simulink model "Copy_of_sistema_angulo"  (R2024b)
settings: Solver=ode4  StartTime=0.0  StopTime=tfin+ts  FixedStep=ts  MaxStep=ts  RelTol=1e-6  AbsTol=1e-9
values from neighbouring files (symbols this model uses):
  alfaini = 0    [Ensayo 9_2.mat]    (also in Ensayo_7_3.mat; Ensayo_8_3.mat; prep_datos_angulo.m)
  Kinterno = 80    [Ensayo 9_2.mat]    (also in EnsayoRobot.m = 100; Ensayo_7_3.mat; Ensayo_8_3.mat; parametros_simulink_5_2_1.m)
  th = [0.028057 0.15772]    [Ensayo 9_2.mat]    (also in Ensayo1.mat = [0.00207452760074 0.0610946451897 0.07411845842]; Ensayo10.mat = [0.00207452760074 0.0610946451897 0.07411845842]; Ensayo11.mat = [0.00207452760074 0.0610946451897 0.07411845842]; Ensayo2.mat = [0.00207452760074 0.0610946451897 0.07411845842])
settings Model: Creator=zamora  LastModifiedBy=laboratorios
settings SolverCC: AutoScaleAbsTol=off  ZeroCrossAlgorithm=Adaptive  AlgebraicLoopSolver=TrustRegion
settings DataIOCC: SaveFormat=Array  SignalLoggingSaveFormat=ModelDataLogs  SaveOutput=off  SaveTime=off  ReturnWorkspaceOutputs=off  StateSaveName=x  TimeSaveName=t  OutputSaveName=y
settings OptimizationCC: BlockReduction=off  BooleanDataType=off  DefaultParameterBehavior=Inlined  BufferReuse=off  ReuseModelBlockBuffer=off  ExpressionDepthLimit=2147483647  LifeSpan=inf
settings DebuggingCC: SaveWithParameterizedLinksMsg=none  UnderspecifiedInitializationDetection=Classic  MergeDetectMultiDrivingBlocksExec=none  SignalResolutionControl=TryResolveAllWithWarning  MaxConsecutiveZCsMsg=none  IgnoredZcDiagnostic=none  MultiTaskDSMMsg=warning  MultiTaskCondExecSysMsg=none  FcnCallInpInsideContextMsg=warning  UnconnectedInputMsg=warning  UnconnectedOutputMsg=warning  UnconnectedLineMsg=warning  StateNameClashWarn=warning  SFUnexpectedBacktrackingDiag=warning  SFNoUnconditionalDefaultTransitionDiag=warning  SFExecutionAtInitializationDiag=none  ArithmeticOperatorsInVariantConditions=warning
settings HardwareCC: ProdBitPerPointer=32  ProdBitPerSizeT=32  ProdBitPerPtrDiffT=32  ProdLargestAtomicFloat=None  ProdIntDivRoundTo=Undefined  ProdEndianess=Unspecified  ProdWordSize=32  ProdHWDeviceType=32-bit Generic  TargetUnknown=on
settings ModelReferenceCC: EnableRefExpFcnMdlSchedulingChecks=on  PropagateSignalLabelsOutOfModel=off
settings SFSimCC: SimUseLocalCustomCode=off  CustomCodeUndefinedFunction=UseInterfaceOnly
settings RTWCC: TemplateMakefile=grt_unix.tmf  RTWUseLocalCustomCode=off  GPUComputeCapability=3.5
settings CodeAppCC: StateflowObjectComments=on
settings GRTTargetCC: TargetLangStandard=C89/C90 (ANSI)  CombineOutputUpdateFcns=off  GRTInterface=on
settings ConfigComp: CovMetricSettings=dw  CovSaveCumulativeToWorkspaceVar=on  CovSaveSingleToWorkspaceVar=on  CovExternalEMLEnable=off  CovSFcnEnable=off

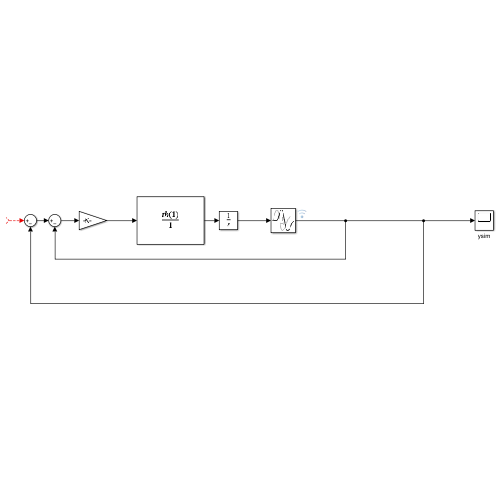
[thumbnail: Simulink's stored preview of the top-level diagram]
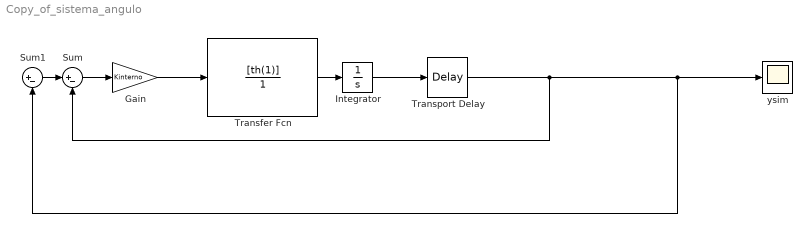
== system Copy_of_sistema_angulo ==
  Gain : Gain  Gain=Kinterno
  Integrator : Integrator  InitialCondition=alfaini
  Sum : Sum  Inputs=|+-
  Sum1 : Sum  Inputs=|+-
  Transfer Fcn : TransferFcn  Numerator=[th(1)]  Denominator=[0 1]
  Transport Delay : TransportDelay  DelayTime=th(2)
  ysim : Scope
  wires:
  Sum/1 -> Gain/1
  Transfer Fcn/1 -> Integrator/1
  Integrator/1 -> Transport Delay/1
  Gain/1 -> Transfer Fcn/1
  Transport Delay/1 -> Sum/2, Sum1/2, ysim/1
  ? -> Sum1/1
  Sum1/1 -> Sum/1
